simulink model "sm_car_"  (R2026b)
settings: Solver=ode23t  StopTime=100  MaxStep=0.4  AbsTol=1e-3  EnableMultiTasking=on
PreLoadFcn:
  | % Due to usability issue in Repeating Sequence block
  | warning('off','Simulink:Masking:Invalid');
  | 
  | % Eliminate unnecessary warnings in inactive variants
  | % Warnings generated only if you click through inactive variant
  | warning('off','MATLAB:nonExistentField');
  | warning('off','Simulink:Parameters:BlkParamUndefined');
PostLoadFcn:
  | set_param([bdroot '/Vehicle'],'popup_trailer','Off')
  | warning('off','sm:sli:setup:compile:LocalSolverNotSupported')
  | %sm_car_config_maneuver(bdroot,'WOT Braking');
  | sm_car_config_vehicle(bdroot,'false');
  | sm_car_config_logging(bdroot);
InitFcn:
  | sm_car_config_camera;
  | Vehicle = sm_car_vehcfg_checkConfig(Vehicle);
  | sm_car_check_tire_model(bdroot);
StartFcn:
  | tic;
StopFcn:
  | Elapsed_Sim_Time = toc;
  | % disp(['Elapsed Sim Time = ' num2str(Elapsed_Sim_Time)]);
undefined symbols (not defined in the file or in its folder): acc_theta, accel_ramp_rate, Axle1D, AxleIn, Camera, Control, Driver, Init, Maneuver, Pedal, Scene, ShaftL1, ShaftL2, ShaftR1, ShaftR2, Visual, X, xy_data_car_side, Y, Z
libraries: sm_lib x290, fl_lib x171, nesl_utility x144, simulink x60, simulink_extras x14, sdl_lib x14, SimscapeFluids_lib x7, Damper_Element x4, Tire_1x2x x4, ee_lib x3, Scene_Utilities x3, sharedTrackingLibrary x2
(part 7 of 22)

== system sm_car_/Vehicle/Trailer/None ==
  note: Ports deliberately not connected. They are necessary for unit tests, but not necessary here.
  "RdBus " : Inport
  "DrvBus " : Inport  Port=2
  "CtrlBus " : Inport  Port=3
  Ground : Ground
  Reference Frame : sm_lib/Frames and Transforms/Reference Frame
  Terminator : Terminator
  Terminator1 : Terminator
  Terminator2 : Terminator
  " C" : PMIOPort  Side=Left
  " W" : PMIOPort  Port=2  Side=Left
  " Hitch" : PMIOPort  Port=3  Side=Right
  " VehBus" : Outport  VectorParamsAs1DForOutWhenUnconnected=off
  wires:
  "RdBus "/1 -> Terminator/1
  "DrvBus "/1 -> Terminator1/1
  "CtrlBus "/1 -> Terminator2/1
  Ground/1 -> " VehBus"/1
  connections:
  " Hitch"/RConn1 -- Reference Frame/RConn1

== system sm_car_/Vehicle/Vehicle/A1 to World ==
  Body World Joint : sm_lib/Joints/6-DOF Joint  JointMode=Normal  CompositeWrenchDir=FollowerOnBase  CompositeWrenchFrame=BaseFrame  SenseConstraintForce=off  SenseConstraintTorque=off  SenseTotalForce=off  SenseTotalTorque=off  PxPositionTargetSpecify=off  PxPositionTargetPriority=Low  PxPositionTargetValue=Init.sChassis.Value(1)  PxPositionTargetValueUnits=m  PxVelocityTargetSpecify=off  PxVelocityTargetPriority=Low  PxVelocityTargetValue=initial_vveh(1)  PxVelocityTargetValueUnits=m/s  PxEquilibriumPosition=0  PxEquilibriumPositionUnits=m  PxSpringStiffness=0  PxSpringStiffnessUnits=N/m  PxDampingCoefficient=0  PxDampingCoefficientUnits=N/(m/s)  PxLowerLimitSpecify=off  PxLowerLimitBound=-1  PxLowerLimitBoundUnits=m  PxLowerLimitStiffness=1e6  PxLowerLimitStiffnessUnits=N/m  PxLowerLimitDamping=1e3  PxLowerLimitDampingUnits=N/(m/s)  PxLowerLimitTransitionRegionWidth=1e-4  PxLowerLimitTransitionRegionWidthUnits=m  PxUpperLimitSpecify=off  PxUpperLimitBound=1  PxUpperLimitBoundUnits=m  PxUpperLimitStiffness=1e6  PxUpperLimitStiffnessUnits=N/m  PxUpperLimitDamping=1e3  PxUpperLimitDampingUnits=N/(m/s)  PxUpperLimitTransitionRegionWidth=1e-4  PxUpperLimitTransitionRegionWidthUnits=m  PxTorqueActuationMode=NoTorque  PxMotionActuationMode=ComputedMotion  PxSensePosition=off  PxSenseVelocity=off  PxSenseAcceleration=off  PxSenseTorqueForce=off  PxSenseLowerLimitTorqueForce=off  PxSenseUpperLimitTorqueForce=off  PyPositionTargetSpecify=off  PyPositionTargetPriority=Low  PyPositionTargetValue=Init.sChassis.Value(2)  PyPositionTargetValueUnits=m  PyVelocityTargetSpecify=off  PyVelocityTargetPriority=Low  PyVelocityTargetValue=initial_vveh(2)  PyVelocityTargetValueUnits=m/s  PyEquilibriumPosition=0  PyEquilibriumPositionUnits=m  PySpringStiffness=0  PySpringStiffnessUnits=N/m  PyDampingCoefficient=0  PyDampingCoefficientUnits=N/(m/s)  PyLowerLimitSpecify=off  PyLowerLimitBound=-1  PyLowerLimitBoundUnits=m  PyLowerLimitStiffness=1e6  PyLowerLimitStiffnessUnits=N/m  PyLowerLimitDamping=1e3  PyLowerLimitDampingUnits=N/(m/s)  PyLowerLimitTransitionRegionWidth=1e-4  PyLowerLimitTransitionRegionWidthUnits=m  PyUpperLimitSpecify=off  PyUpperLimitBound=1  PyUpperLimitBoundUnits=m  PyUpperLimitStiffness=1e6  PyUpperLimitStiffnessUnits=N/m  PyUpperLimitDamping=1e3  PyUpperLimitDampingUnits=N/(m/s)  PyUpperLimitTransitionRegionWidth=1e-4  PyUpperLimitTransitionRegionWidthUnits=m  PyTorqueActuationMode=NoTorque  PyMotionActuationMode=ComputedMotion  PySensePosition=off  PySenseVelocity=off  PySenseAcceleration=off  PySenseTorqueForce=off  PySenseLowerLimitTorqueForce=off  PySenseUpperLimitTorqueForce=off  PzPositionTargetSpecify=off  PzPositionTargetPriority=Low  PzPositionTargetValue=Init.sChassis.Value(3)  PzPositionTargetValueUnits=m  PzVelocityTargetSpecify=off  PzVelocityTargetPriority=Low  PzVelocityTargetValue=initial_vveh(3)  PzVelocityTargetValueUnits=m/s  PzEquilibriumPosition=0  PzEquilibriumPositionUnits=m  PzSpringStiffness=0  PzSpringStiffnessUnits=N/m  PzDampingCoefficient=0  PzDampingCoefficientUnits=N/(m/s)  PzLowerLimitSpecify=off  PzLowerLimitBound=-1  PzLowerLimitBoundUnits=m  PzLowerLimitStiffness=1e6  PzLowerLimitStiffnessUnits=N/m  PzLowerLimitDamping=1e3  PzLowerLimitDampingUnits=N/(m/s)  PzLowerLimitTransitionRegionWidth=1e-4  PzLowerLimitTransitionRegionWidthUnits=m  PzUpperLimitSpecify=off  PzUpperLimitBound=1  PzUpperLimitBoundUnits=m  PzUpperLimitStiffness=1e6  PzUpperLimitStiffnessUnits=N/m  PzUpperLimitDamping=1e3  PzUpperLimitDampingUnits=N/(m/s)  PzUpperLimitTransitionRegionWidth=1e-4  PzUpperLimitTransitionRegionWidthUnits=m  PzTorqueActuationMode=NoTorque  PzMotionActuationMode=ComputedMotion  PzSensePosition=on  PzSenseVelocity=off  PzSenseAcceleration=off  PzSenseTorqueForce=off  PzSenseLowerLimitTorqueForce=off  PzSenseUpperLimitTorqueForce=off  SphPositionTargetSpecify=off  SphPositionTargetPriority=Low  SphPositionTargetRotationMethod=RotationSequence  SphPositionTargetFollAlignAxisA=+X  SphPositionTargetBaseAlignAxisA=+Y  SphPositionTargetFollAlignAxisB=+Y  SphPositionTargetBaseAlignAxisB=+Z  SphPositionTargetRotationStandardAxis=+Z  SphPositionTargetRotationAngle=0.0  SphPositionTargetRotationAngleUnits=deg  SphPositionTargetRotationArbitraryAxis=[0 0 1]  SphPositionTargetRotationSequenceAxes=FollowerAxes  SphPositionTargetRotationSequence=ZYX  SphPositionTargetRotationSequenceAngles=initial_aveh  SphPositionTargetRotationSequenceAnglesUnits=rad  SphPositionTargetRotationMatrix=[1 0 0; 0 1 0; 0 0 1]  SphPositionTargetQuaternion=[1 0 0 0]  SphVelocityTargetSpecify=off  SphVelocityTargetPriority=High  SphVelocityTargetValue=[0 0 0]  SphVelocityTargetValueUnits=deg/s  SphVelocityTargetInFollowerFrame=on  SphEqPosRotationMethod=None  SphEqPosFollAlignAxisA=+X  SphEqPosBaseAlignAxisA=+Y  SphEqPosFollAlignAxisB=+Y  SphEqPosBaseAlignAxisB=+Z  SphEqPosRotationStandardAxis=+Z  SphEqPosRotationAngle=0.0  SphEqPosRotationAngleUnits=deg  SphEqPosRotationArbitraryAxis=[0 0 1]  SphEqPosRotationSequenceAxes=FollowerAxes  SphEqPosRotationSequence=XYX  SphEqPosRotationSequenceAngles=[0 0 0]  SphEqPosRotationSequenceAnglesUnits=deg  SphEqPosRotationMatrix=[1 0 0; 0 1 0; 0 0 1]  SphEqPosQuaternion=[1 0 0 0]  SphSpringStiffness=0  SphSpringStiffnessUnits=N*m/deg  SphDampingCoefficient=0  SphDampingCoefficientUnits=N*m/(deg/s)  SphLowerLimitSpecify=off  SphLowerLimitBound=15  SphLowerLimitBoundUnits=deg  SphLowerLimitStiffness=1e4  SphLowerLimitStiffnessUnits=N*m/deg  SphLowerLimitDamping=10  SphLowerLimitDampingUnits=N*m/(deg/s)  SphLowerLimitTransitionRegionWidth=0.1  SphLowerLimitTransitionRegionWidthUnits=deg  SphUpperLimitSpecify=off  SphUpperLimitBound=45  SphUpperLimitBoundUnits=deg  SphUpperLimitStiffness=1e4  SphUpperLimitStiffnessUnits=N*m/deg  SphUpperLimitDamping=10  SphUpperLimitDampingUnits=N*m/(deg/s)  SphUpperLimitTransitionRegionWidth=0.1  SphUpperLimitTransitionRegionWidthUnits=deg  SphTorqueActuationMode=NoTorque  SphActuateTorqueX=off  SphActuateTorqueY=off  SphActuateTorqueZ=off  SphActuateTorque=off  SphActuationFrame=BaseFrame  SphSensePosition=off  SphSenseVelocityX=off  SphSenseVelocityY=off  SphSenseVelocityZ=off  SphSenseVelocity=off  SphSenseAccelerationX=off  SphSenseAccelerationY=off  SphSenseAccelerationZ=off  SphSenseAcceleration=off  SphSenseLowerLimitTorqueMag=off  SphSenseUpperLimitTorqueMag=off  SphSensingFrame=BaseFrame
  PS-Simulink Converter2 : nesl_utility/PS-Simulink Converter  PhysicalDomain=network_engine_domain  SubClassName=ps_output  LeftPortType=input  RightPortType=output  PseudoPeriodic=off  Frequencies=[]  VectorFormat=1-D array  Unit=m  AffineConversion=off
  Transform Sensor : sm_lib/Frames and Transforms/Transform Sensor  ObservationFrame=World  ExpressedInFrame=World  RotationSequence=XYX  SenseAngle=off  SenseAxis=off  SenseQ=off  SenseR=off  SenseRotationSequence=off  SenseOmegaX=off  SenseOmegaY=off  SenseOmegaZ=off  SenseOmega=off  SenseQDot=off  SenseRDot=off  SenseRotationSequenceDot=off  SenseAlphaX=off  SenseAlphaY=off  SenseAlphaZ=off  SenseAlpha=off  SenseQDDot=off  SenseRDDot=off  SenseX=off  SenseY=off  SenseZ=off  SenseXYZ=off  SenseRad=off  SenseAzim=off  SenseDist=off  SenseInc=off  SenseXDot=off  SenseYDot=off  SenseZDot=off  SenseXYZDot=off  SenseRadDot=off  SenseAzimDot=off  SenseDistDot=off  SenseIncDot=off  SenseXDDot=off  SenseYDDot=off  SenseZDDot=off  SenseXYZDDot=off  SenseRadDDot=off  SenseAzimDDot=off  SenseDistDDot=off  SenseIncDDot=off
  F : PMIOPort  Side=Left
  B : PMIOPort  Port=2  Side=Right
  Bus Element Out6 : Outport  VectorParamsAs1DForOutWhenUnconnected=off  PortName=World  Element=z
  wires:
  PS-Simulink Converter2/1 -> Bus Element Out6/1
  connections:
  Body World Joint/RConn2 -- PS-Simulink Converter2/LConn1
  Body World Joint/RConn1 -- F/RConn1 -- Transform Sensor/RConn1
  Body World Joint/LConn1 -- B/RConn1 -- Transform Sensor/LConn1

== system sm_car_/Vehicle/Vehicle/A2 to World ==
  Body World Joint : sm_lib/Joints/6-DOF Joint  JointMode=Normal  CompositeWrenchDir=FollowerOnBase  CompositeWrenchFrame=BaseFrame  SenseConstraintForce=off  SenseConstraintTorque=off  SenseTotalForce=off  SenseTotalTorque=off  PxPositionTargetSpecify=off  PxPositionTargetPriority=Low  PxPositionTargetValue=Init.sChassis.Value(1)  PxPositionTargetValueUnits=m  PxVelocityTargetSpecify=off  PxVelocityTargetPriority=Low  PxVelocityTargetValue=initial_vveh(1)  PxVelocityTargetValueUnits=m/s  PxEquilibriumPosition=0  PxEquilibriumPositionUnits=m  PxSpringStiffness=0  PxSpringStiffnessUnits=N/m  PxDampingCoefficient=0  PxDampingCoefficientUnits=N/(m/s)  PxLowerLimitSpecify=off  PxLowerLimitBound=-1  PxLowerLimitBoundUnits=m  PxLowerLimitStiffness=1e6  PxLowerLimitStiffnessUnits=N/m  PxLowerLimitDamping=1e3  PxLowerLimitDampingUnits=N/(m/s)  PxLowerLimitTransitionRegionWidth=1e-4  PxLowerLimitTransitionRegionWidthUnits=m  PxUpperLimitSpecify=off  PxUpperLimitBound=1  PxUpperLimitBoundUnits=m  PxUpperLimitStiffness=1e6  PxUpperLimitStiffnessUnits=N/m  PxUpperLimitDamping=1e3  PxUpperLimitDampingUnits=N/(m/s)  PxUpperLimitTransitionRegionWidth=1e-4  PxUpperLimitTransitionRegionWidthUnits=m  PxTorqueActuationMode=NoTorque  PxMotionActuationMode=ComputedMotion  PxSensePosition=off  PxSenseVelocity=off  PxSenseAcceleration=off  PxSenseTorqueForce=off  PxSenseLowerLimitTorqueForce=off  PxSenseUpperLimitTorqueForce=off  PyPositionTargetSpecify=off  PyPositionTargetPriority=Low  PyPositionTargetValue=Init.sChassis.Value(2)  PyPositionTargetValueUnits=m  PyVelocityTargetSpecify=off  PyVelocityTargetPriority=Low  PyVelocityTargetValue=initial_vveh(2)  PyVelocityTargetValueUnits=m/s  PyEquilibriumPosition=0  PyEquilibriumPositionUnits=m  PySpringStiffness=0  PySpringStiffnessUnits=N/m  PyDampingCoefficient=0  PyDampingCoefficientUnits=N/(m/s)  PyLowerLimitSpecify=off  PyLowerLimitBound=-1  PyLowerLimitBoundUnits=m  PyLowerLimitStiffness=1e6  PyLowerLimitStiffnessUnits=N/m  PyLowerLimitDamping=1e3  PyLowerLimitDampingUnits=N/(m/s)  PyLowerLimitTransitionRegionWidth=1e-4  PyLowerLimitTransitionRegionWidthUnits=m  PyUpperLimitSpecify=off  PyUpperLimitBound=1  PyUpperLimitBoundUnits=m  PyUpperLimitStiffness=1e6  PyUpperLimitStiffnessUnits=N/m  PyUpperLimitDamping=1e3  PyUpperLimitDampingUnits=N/(m/s)  PyUpperLimitTransitionRegionWidth=1e-4  PyUpperLimitTransitionRegionWidthUnits=m  PyTorqueActuationMode=NoTorque  PyMotionActuationMode=ComputedMotion  PySensePosition=off  PySenseVelocity=off  PySenseAcceleration=off  PySenseTorqueForce=off  PySenseLowerLimitTorqueForce=off  PySenseUpperLimitTorqueForce=off  PzPositionTargetSpecify=off  PzPositionTargetPriority=Low  PzPositionTargetValue=Init.sChassis.Value(3)  PzPositionTargetValueUnits=m  PzVelocityTargetSpecify=off  PzVelocityTargetPriority=Low  PzVelocityTargetValue=initial_vveh(3)  PzVelocityTargetValueUnits=m/s  PzEquilibriumPosition=0  PzEquilibriumPositionUnits=m  PzSpringStiffness=0  PzSpringStiffnessUnits=N/m  PzDampingCoefficient=0  PzDampingCoefficientUnits=N/(m/s)  PzLowerLimitSpecify=off  PzLowerLimitBound=-1  PzLowerLimitBoundUnits=m  PzLowerLimitStiffness=1e6  PzLowerLimitStiffnessUnits=N/m  PzLowerLimitDamping=1e3  PzLowerLimitDampingUnits=N/(m/s)  PzLowerLimitTransitionRegionWidth=1e-4  PzLowerLimitTransitionRegionWidthUnits=m  PzUpperLimitSpecify=off  PzUpperLimitBound=1  PzUpperLimitBoundUnits=m  PzUpperLimitStiffness=1e6  PzUpperLimitStiffnessUnits=N/m  PzUpperLimitDamping=1e3  PzUpperLimitDampingUnits=N/(m/s)  PzUpperLimitTransitionRegionWidth=1e-4  PzUpperLimitTransitionRegionWidthUnits=m  PzTorqueActuationMode=NoTorque  PzMotionActuationMode=ComputedMotion  PzSensePosition=on  PzSenseVelocity=off  PzSenseAcceleration=off  PzSenseTorqueForce=off  PzSenseLowerLimitTorqueForce=off  PzSenseUpperLimitTorqueForce=off  SphPositionTargetSpecify=off  SphPositionTargetPriority=Low  SphPositionTargetRotationMethod=RotationSequence  SphPositionTargetFollAlignAxisA=+X  SphPositionTargetBaseAlignAxisA=+Y  SphPositionTargetFollAlignAxisB=+Y  SphPositionTargetBaseAlignAxisB=+Z  SphPositionTargetRotationStandardAxis=+Z  SphPositionTargetRotationAngle=0.0  SphPositionTargetRotationAngleUnits=deg  SphPositionTargetRotationArbitraryAxis=[0 0 1]  SphPositionTargetRotationSequenceAxes=FollowerAxes  SphPositionTargetRotationSequence=ZYX  SphPositionTargetRotationSequenceAngles=initial_aveh  SphPositionTargetRotationSequenceAnglesUnits=rad  SphPositionTargetRotationMatrix=[1 0 0; 0 1 0; 0 0 1]  SphPositionTargetQuaternion=[1 0 0 0]  SphVelocityTargetSpecify=off  SphVelocityTargetPriority=High  SphVelocityTargetValue=[0 0 0]  SphVelocityTargetValueUnits=deg/s  SphVelocityTargetInFollowerFrame=on  SphEqPosRotationMethod=None  SphEqPosFollAlignAxisA=+X  SphEqPosBaseAlignAxisA=+Y  SphEqPosFollAlignAxisB=+Y  SphEqPosBaseAlignAxisB=+Z  SphEqPosRotationStandardAxis=+Z  SphEqPosRotationAngle=0.0  SphEqPosRotationAngleUnits=deg  SphEqPosRotationArbitraryAxis=[0 0 1]  SphEqPosRotationSequenceAxes=FollowerAxes  SphEqPosRotationSequence=XYX  SphEqPosRotationSequenceAngles=[0 0 0]  SphEqPosRotationSequenceAnglesUnits=deg  SphEqPosRotationMatrix=[1 0 0; 0 1 0; 0 0 1]  SphEqPosQuaternion=[1 0 0 0]  SphSpringStiffness=0  SphSpringStiffnessUnits=N*m/deg  SphDampingCoefficient=0  SphDampingCoefficientUnits=N*m/(deg/s)  SphLowerLimitSpecify=off  SphLowerLimitBound=15  SphLowerLimitBoundUnits=deg  SphLowerLimitStiffness=1e4  SphLowerLimitStiffnessUnits=N*m/deg  SphLowerLimitDamping=10  SphLowerLimitDampingUnits=N*m/(deg/s)  SphLowerLimitTransitionRegionWidth=0.1  SphLowerLimitTransitionRegionWidthUnits=deg  SphUpperLimitSpecify=off  SphUpperLimitBound=45  SphUpperLimitBoundUnits=deg  SphUpperLimitStiffness=1e4  SphUpperLimitStiffnessUnits=N*m/deg  SphUpperLimitDamping=10  SphUpperLimitDampingUnits=N*m/(deg/s)  SphUpperLimitTransitionRegionWidth=0.1  SphUpperLimitTransitionRegionWidthUnits=deg  SphTorqueActuationMode=NoTorque  SphActuateTorqueX=off  SphActuateTorqueY=off  SphActuateTorqueZ=off  SphActuateTorque=off  SphActuationFrame=BaseFrame  SphSensePosition=off  SphSenseVelocityX=off  SphSenseVelocityY=off  SphSenseVelocityZ=off  SphSenseVelocity=off  SphSenseAccelerationX=off  SphSenseAccelerationY=off  SphSenseAccelerationZ=off  SphSenseAcceleration=off  SphSenseLowerLimitTorqueMag=off  SphSenseUpperLimitTorqueMag=off  SphSensingFrame=BaseFrame
  PS-Simulink Converter2 : nesl_utility/PS-Simulink Converter  PhysicalDomain=network_engine_domain  SubClassName=ps_output  LeftPortType=input  RightPortType=output  PseudoPeriodic=off  Frequencies=[]  VectorFormat=1-D array  Unit=m  AffineConversion=off
  Transform Sensor : sm_lib/Frames and Transforms/Transform Sensor  ObservationFrame=World  ExpressedInFrame=World  RotationSequence=XYX  SenseAngle=off  SenseAxis=off  SenseQ=off  SenseR=off  SenseRotationSequence=off  SenseOmegaX=off  SenseOmegaY=off  SenseOmegaZ=off  SenseOmega=off  SenseQDot=off  SenseRDot=off  SenseRotationSequenceDot=off  SenseAlphaX=off  SenseAlphaY=off  SenseAlphaZ=off  SenseAlpha=off  SenseQDDot=off  SenseRDDot=off  SenseX=off  SenseY=off  SenseZ=off  SenseXYZ=off  SenseRad=off  SenseAzim=off  SenseDist=off  SenseInc=off  SenseXDot=off  SenseYDot=off  SenseZDot=off  SenseXYZDot=off  SenseRadDot=off  SenseAzimDot=off  SenseDistDot=off  SenseIncDot=off  SenseXDDot=off  SenseYDDot=off  SenseZDDot=off  SenseXYZDDot=off  SenseRadDDot=off  SenseAzimDDot=off  SenseDistDDot=off  SenseIncDDot=off
  F : PMIOPort  Side=Left
  B : PMIOPort  Port=2  Side=Right
  Bus Element Out6 : Outport  VectorParamsAs1DForOutWhenUnconnected=off  PortName=World  Element=z
  wires:
  PS-Simulink Converter2/1 -> Bus Element Out6/1
  connections:
  B/RConn1 -- Transform Sensor/LConn1 -- Body World Joint/LConn1
  Body World Joint/RConn1 -- Transform Sensor/RConn1 -- F/RConn1
  Body World Joint/RConn2 -- PS-Simulink Converter2/LConn1

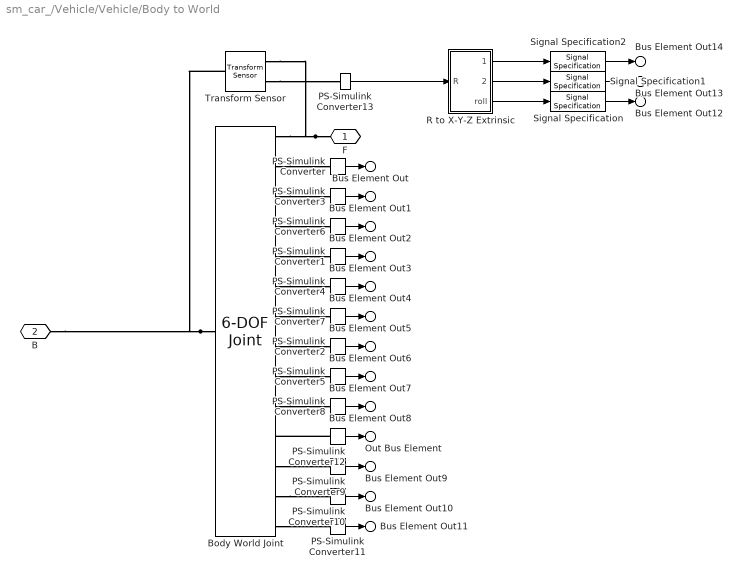
== system sm_car_/Vehicle/Vehicle/Body to World ==
  Body World Joint : sm_lib/Joints/6-DOF Joint  JointMode=Normal  CompositeWrenchDir=FollowerOnBase  CompositeWrenchFrame=BaseFrame  SenseConstraintForce=off  SenseConstraintTorque=off  SenseTotalForce=off  SenseTotalTorque=off  PxPositionTargetSpecify=on  PxPositionTargetPriority=Low  PxPositionTargetValue=Init.sChassis.Value(1)  PxPositionTargetValueUnits=m  PxVelocityTargetSpecify=on  PxVelocityTargetPriority=Low  PxVelocityTargetValue=initial_vveh(1)  PxVelocityTargetValueUnits=m/s  PxEquilibriumPosition=0  PxEquilibriumPositionUnits=m  PxSpringStiffness=0  PxSpringStiffnessUnits=N/m  PxDampingCoefficient=0  PxDampingCoefficientUnits=N/(m/s)  PxLowerLimitSpecify=off  PxLowerLimitBound=-1  PxLowerLimitBoundUnits=m  PxLowerLimitStiffness=1e6  PxLowerLimitStiffnessUnits=N/m  PxLowerLimitDamping=1e3  PxLowerLimitDampingUnits=N/(m/s)  PxLowerLimitTransitionRegionWidth=1e-4  PxLowerLimitTransitionRegionWidthUnits=m  PxUpperLimitSpecify=off  PxUpperLimitBound=1  PxUpperLimitBoundUnits=m  PxUpperLimitStiffness=1e6  PxUpperLimitStiffnessUnits=N/m  PxUpperLimitDamping=1e3  PxUpperLimitDampingUnits=N/(m/s)  PxUpperLimitTransitionRegionWidth=1e-4  PxUpperLimitTransitionRegionWidthUnits=m  PxTorqueActuationMode=NoTorque  PxMotionActuationMode=ComputedMotion  PxSensePosition=on  PxSenseVelocity=on  PxSenseAcceleration=on  PxSenseTorqueForce=off  PxSenseLowerLimitTorqueForce=off  PxSenseUpperLimitTorqueForce=off  PyPositionTargetSpecify=on  PyPositionTargetPriority=Low  PyPositionTargetValue=Init.sChassis.Value(2)  PyPositionTargetValueUnits=m  PyVelocityTargetSpecify=on  PyVelocityTargetPriority=Low  PyVelocityTargetValue=initial_vveh(2)  PyVelocityTargetValueUnits=m/s  PyEquilibriumPosition=0  PyEquilibriumPositionUnits=m  PySpringStiffness=0  PySpringStiffnessUnits=N/m  PyDampingCoefficient=0  PyDampingCoefficientUnits=N/(m/s)  PyLowerLimitSpecify=off  PyLowerLimitBound=-1  PyLowerLimitBoundUnits=m  PyLowerLimitStiffness=1e6  PyLowerLimitStiffnessUnits=N/m  PyLowerLimitDamping=1e3  PyLowerLimitDampingUnits=N/(m/s)  PyLowerLimitTransitionRegionWidth=1e-4  PyLowerLimitTransitionRegionWidthUnits=m  PyUpperLimitSpecify=off  PyUpperLimitBound=1  PyUpperLimitBoundUnits=m  PyUpperLimitStiffness=1e6  PyUpperLimitStiffnessUnits=N/m  PyUpperLimitDamping=1e3  PyUpperLimitDampingUnits=N/(m/s)  PyUpperLimitTransitionRegionWidth=1e-4  PyUpperLimitTransitionRegionWidthUnits=m  PyTorqueActuationMode=NoTorque  PyMotionActuationMode=ComputedMotion  PySensePosition=on  PySenseVelocity=on  PySenseAcceleration=on  PySenseTorqueForce=off  PySenseLowerLimitTorqueForce=off  PySenseUpperLimitTorqueForce=off  PzPositionTargetSpecify=on  PzPositionTargetPriority=Low  PzPositionTargetValue=Init.sChassis.Value(3)  PzPositionTargetValueUnits=m  PzVelocityTargetSpecify=on  PzVelocityTargetPriority=Low  PzVelocityTargetValue=initial_vveh(3)  PzVelocityTargetValueUnits=m/s  PzEquilibriumPosition=0  PzEquilibriumPositionUnits=m  PzSpringStiffness=0  PzSpringStiffnessUnits=N/m  PzDampingCoefficient=0  PzDampingCoefficientUnits=N/(m/s)  PzLowerLimitSpecify=off  PzLowerLimitBound=-1  PzLowerLimitBoundUnits=m  PzLowerLimitStiffness=1e6  PzLowerLimitStiffnessUnits=N/m  PzLowerLimitDamping=1e3  PzLowerLimitDampingUnits=N/(m/s)  PzLowerLimitTransitionRegionWidth=1e-4  PzLowerLimitTransitionRegionWidthUnits=m  PzUpperLimitSpecify=off  PzUpperLimitBound=1  PzUpperLimitBoundUnits=m  PzUpperLimitStiffness=1e6  PzUpperLimitStiffnessUnits=N/m  PzUpperLimitDamping=1e3  PzUpperLimitDampingUnits=N/(m/s)  PzUpperLimitTransitionRegionWidth=1e-4  PzUpperLimitTransitionRegionWidthUnits=m  PzTorqueActuationMode=NoTorque  PzMotionActuationMode=ComputedMotion  PzSensePosition=on  PzSenseVelocity=on  PzSenseAcceleration=on  PzSenseTorqueForce=off  PzSenseLowerLimitTorqueForce=off  PzSenseUpperLimitTorqueForce=off  SphPositionTargetSpecify=on  SphPositionTargetPriority=Low  SphPositionTargetRotationMethod=RotationSequence  SphPositionTargetFollAlignAxisA=+X  SphPositionTargetBaseAlignAxisA=+Y  SphPositionTargetFollAlignAxisB=+Y  SphPositionTargetBaseAlignAxisB=+Z  SphPositionTargetRotationStandardAxis=+Z  SphPositionTargetRotationAngle=0.0  SphPositionTargetRotationAngleUnits=deg  SphPositionTargetRotationArbitraryAxis=[0 0 1]  SphPositionTargetRotationSequenceAxes=FollowerAxes  SphPositionTargetRotationSequence=ZYX  SphPositionTargetRotationSequenceAngles=initial_aveh  SphPositionTargetRotationSequenceAnglesUnits=rad  SphPositionTargetRotationMatrix=[1 0 0; 0 1 0; 0 0 1]  SphPositionTargetQuaternion=[1 0 0 0]  SphVelocityTargetSpecify=off  SphVelocityTargetPriority=High  SphVelocityTargetValue=[0 0 0]  SphVelocityTargetValueUnits=deg/s  SphVelocityTargetInFollowerFrame=on  SphEqPosRotationMethod=None  SphEqPosFollAlignAxisA=+X  SphEqPosBaseAlignAxisA=+Y  SphEqPosFollAlignAxisB=+Y  SphEqPosBaseAlignAxisB=+Z  SphEqPosRotationStandardAxis=+Z  SphEqPosRotationAngle=0.0  SphEqPosRotationAngleUnits=deg  SphEqPosRotationArbitraryAxis=[0 0 1]  SphEqPosRotationSequenceAxes=FollowerAxes  SphEqPosRotationSequence=XYX  SphEqPosRotationSequenceAngles=[0 0 0]  SphEqPosRotationSequenceAnglesUnits=deg  SphEqPosRotationMatrix=[1 0 0; 0 1 0; 0 0 1]  SphEqPosQuaternion=[1 0 0 0]  SphSpringStiffness=0  SphSpringStiffnessUnits=N*m/deg  SphDampingCoefficient=0  SphDampingCoefficientUnits=N*m/(deg/s)  SphLowerLimitSpecify=off  SphLowerLimitBound=15  SphLowerLimitBoundUnits=deg  SphLowerLimitStiffness=1e4  SphLowerLimitStiffnessUnits=N*m/deg  SphLowerLimitDamping=10  SphLowerLimitDampingUnits=N*m/(deg/s)  SphLowerLimitTransitionRegionWidth=0.1  SphLowerLimitTransitionRegionWidthUnits=deg  SphUpperLimitSpecify=off  SphUpperLimitBound=45  SphUpperLimitBoundUnits=deg  SphUpperLimitStiffness=1e4  SphUpperLimitStiffnessUnits=N*m/deg  SphUpperLimitDamping=10  SphUpperLimitDampingUnits=N*m/(deg/s)  SphUpperLimitTransitionRegionWidth=0.1  SphUpperLimitTransitionRegionWidthUnits=deg  SphTorqueActuationMode=NoTorque  SphActuateTorqueX=off  SphActuateTorqueY=off  SphActuateTorqueZ=off  SphActuateTorque=off  SphActuationFrame=BaseFrame  SphSensePosition=on  SphSenseVelocityX=on  SphSenseVelocityY=on  SphSenseVelocityZ=on  SphSenseVelocity=off  SphSenseAccelerationX=off  SphSenseAccelerationY=off  SphSenseAccelerationZ=off  SphSenseAcceleration=off  SphSenseLowerLimitTorqueMag=off  SphSenseUpperLimitTorqueMag=off  SphSensingFrame=BaseFrame
  PS-Simulink Converter : nesl_utility/PS-Simulink Converter  PhysicalDomain=network_engine_domain  SubClassName=ps_output  LeftPortType=input  RightPortType=output  PseudoPeriodic=off  Frequencies=[]  VectorFormat=1-D array  Unit=m  AffineConversion=off
  PS-Simulink Converter1 : nesl_utility/PS-Simulink Converter  PhysicalDomain=network_engine_domain  SubClassName=ps_output  LeftPortType=input  RightPortType=output  PseudoPeriodic=off  Frequencies=[]  VectorFormat=1-D array  Unit=m  AffineConversion=off
  PS-Simulink Converter10 : nesl_utility/PS-Simulink Converter  PhysicalDomain=network_engine_domain  SubClassName=ps_output  LeftPortType=input  RightPortType=output  PseudoPeriodic=off  Frequencies=[]  VectorFormat=1-D array  Unit=rad/s  AffineConversion=off
  PS-Simulink Converter11 : nesl_utility/PS-Simulink Converter  PhysicalDomain=network_engine_domain  SubClassName=ps_output  LeftPortType=input  RightPortType=output  PseudoPeriodic=off  Frequencies=[]  VectorFormat=1-D array  Unit=rad/s  AffineConversion=off
  PS-Simulink Converter12 : nesl_utility/PS-Simulink Converter  PhysicalDomain=network_engine_domain  SubClassName=ps_output  LeftPortType=input  RightPortType=output  PseudoPeriodic=off  Frequencies=[]  VectorFormat=1-D array  Unit=1  AffineConversion=off
  PS-Simulink Converter13 : nesl_utility/PS-Simulink Converter  PhysicalDomain=network_engine_domain  SubClassName=ps_output  LeftPortType=input  RightPortType=output  PseudoPeriodic=off  Frequencies=[]  VectorFormat=1-D array  Unit=1  AffineConversion=off
  PS-Simulink Converter2 : nesl_utility/PS-Simulink Converter  PhysicalDomain=network_engine_domain  SubClassName=ps_output  LeftPortType=input  RightPortType=output  PseudoPeriodic=off  Frequencies=[]  VectorFormat=1-D array  Unit=m  AffineConversion=off
  PS-Simulink Converter3 : nesl_utility/PS-Simulink Converter  PhysicalDomain=network_engine_domain  SubClassName=ps_output  LeftPortType=input  RightPortType=output  PseudoPeriodic=off  Frequencies=[]  VectorFormat=1-D array  Unit=m/s  AffineConversion=off
  PS-Simulink Converter4 : nesl_utility/PS-Simulink Converter  PhysicalDomain=network_engine_domain  SubClassName=ps_output  LeftPortType=input  RightPortType=output  PseudoPeriodic=off  Frequencies=[]  VectorFormat=1-D array  Unit=m/s  AffineConversion=off
  PS-Simulink Converter5 : nesl_utility/PS-Simulink Converter  PhysicalDomain=network_engine_domain  SubClassName=ps_output  LeftPortType=input  RightPortType=output  PseudoPeriodic=off  Frequencies=[]  VectorFormat=1-D array  Unit=m/s  AffineConversion=off
  PS-Simulink Converter6 : nesl_utility/PS-Simulink Converter  PhysicalDomain=network_engine_domain  SubClassName=ps_output  LeftPortType=input  RightPortType=output  PseudoPeriodic=off  Frequencies=[]  VectorFormat=1-D array  Unit=m/s^2  AffineConversion=off
  PS-Simulink Converter7 : nesl_utility/PS-Simulink Converter  PhysicalDomain=network_engine_domain  SubClassName=ps_output  LeftPortType=input  RightPortType=output  PseudoPeriodic=off  Frequencies=[]  VectorFormat=1-D array  Unit=m/s^2  AffineConversion=off
  PS-Simulink Converter8 : nesl_utility/PS-Simulink Converter  PhysicalDomain=network_engine_domain  SubClassName=ps_output  LeftPortType=input  RightPortType=output  PseudoPeriodic=off  Frequencies=[]  VectorFormat=1-D array  Unit=m/s^2  AffineConversion=off
  PS-Simulink Converter9 : nesl_utility/PS-Simulink Converter  PhysicalDomain=network_engine_domain  SubClassName=ps_output  LeftPortType=input  RightPortType=output  PseudoPeriodic=off  Frequencies=[]  VectorFormat=1-D array  Unit=rad/s  AffineConversion=off
  R to X-Y-Z Extrinsic : Subsystem  mask(Rotation Matrix to X-Y-Z Extrinsic){}
      mask help: Computes roll / pitch / yaw values assuming they correspond to X, Y, and Z rotations, applied in that order and using extrinsic rotations (rotations applied about the fixed axes of the base frame). Does not handle case where Y (pitch) rotation is +/-90 degrees.
  Signal Specification : SignalSpecification  Unit=rad
  Signal Specification1 : SignalSpecification  Unit=rad
  Signal Specification2 : SignalSpecification  Unit=rad
  Transform Sensor : sm_lib/Frames and Transforms/Transform Sensor  ObservationFrame=World  ExpressedInFrame=World  RotationSequence=XYX  SenseAngle=off  SenseAxis=off  SenseQ=off  SenseR=on  SenseRotationSequence=off  SenseOmegaX=off  SenseOmegaY=off  SenseOmegaZ=off  SenseOmega=off  SenseQDot=off  SenseRDot=off  SenseRotationSequenceDot=off  SenseAlphaX=off  SenseAlphaY=off  SenseAlphaZ=off  SenseAlpha=off  SenseQDDot=off  SenseRDDot=off  SenseX=off  SenseY=off  SenseZ=off  SenseXYZ=off  SenseRad=off  SenseAzim=off  SenseDist=off  SenseInc=off  SenseXDot=off  SenseYDot=off  SenseZDot=off  SenseXYZDot=off  SenseRadDot=off  SenseAzimDot=off  SenseDistDot=off  SenseIncDot=off  SenseXDDot=off  SenseYDDot=off  SenseZDDot=off  SenseXYZDDot=off  SenseRadDDot=off  SenseAzimDDot=off  SenseDistDDot=off  SenseIncDDot=off
  F : PMIOPort  Side=Left
  B : PMIOPort  Port=2  Side=Right
  Bus Element Out : Outport  VectorParamsAs1DForOutWhenUnconnected=off  PortName=World  Element=x
  Bus Element Out3 : Outport  VectorParamsAs1DForOutWhenUnconnected=off  PortName=World  Element=y
  Bus Element Out6 : Outport  VectorParamsAs1DForOutWhenUnconnected=off  PortName=World  Element=z
  Bus Element Out1 : Outport  VectorParamsAs1DForOutWhenUnconnected=off  PortName=World  Element=vx
  Bus Element Out4 : Outport  VectorParamsAs1DForOutWhenUnconnected=off  PortName=World  Element=vy
  Bus Element Out7 : Outport  VectorParamsAs1DForOutWhenUnconnected=off  PortName=World  Element=vz
  Bus Element Out2 : Outport  VectorParamsAs1DForOutWhenUnconnected=off  PortName=World  Element=gx
  Bus Element Out5 : Outport  VectorParamsAs1DForOutWhenUnconnected=off  PortName=World  Element=gy
  Bus Element Out8 : Outport  VectorParamsAs1DForOutWhenUnconnected=off  PortName=World  Element=gz
  Bus Element Out9 : Outport  VectorParamsAs1DForOutWhenUnconnected=off  PortName=World  Element=nRoll
  Bus Element Out10 : Outport  VectorParamsAs1DForOutWhenUnconnected=off  PortName=World  Element=nPitch
  Bus Element Out11 : Outport  VectorParamsAs1DForOutWhenUnconnected=off  PortName=World  Element=nYaw
  Bus Element Out12 : Outport  VectorParamsAs1DForOutWhenUnconnected=off  PortName=World  Element=aRoll
  Bus Element Out13 : Outport  VectorParamsAs1DForOutWhenUnconnected=off  PortName=World  Element=aPitch
  Bus Element Out14 : Outport  VectorParamsAs1DForOutWhenUnconnected=off  PortName=World  Element=aYaw
  Out Bus Element : Outport  VectorParamsAs1DForOutWhenUnconnected=off  PortName=World  Element=Q
  wires:
  R to X-Y-Z Extrinsic/1(yaw) -> Signal Specification2/1
  R to X-Y-Z Extrinsic/3(roll) -> Signal Specification/1
  R to X-Y-Z Extrinsic/2(pitch) -> Signal Specification1/1
  PS-Simulink Converter13/1 -> R to X-Y-Z Extrinsic/1(R)
  PS-Simulink Converter12/1 -> Out Bus Element/1
  PS-Simulink Converter11/1 -> Bus Element Out11/1
  PS-Simulink Converter10/1 -> Bus Element Out10/1
  Signal Specification/1 -> Bus Element Out12/1
  Signal Specification1/1 -> Bus Element Out13/1
  Signal Specification2/1 -> Bus Element Out14/1
  PS-Simulink Converter3/1 -> Bus Element Out1/1
  PS-Simulink Converter2/1 -> Bus Element Out6/1
  PS-Simulink Converter6/1 -> Bus Element Out2/1
  PS-Simulink Converter4/1 -> Bus Element Out4/1
  PS-Simulink Converter/1 -> Bus Element Out/1
  PS-Simulink Converter5/1 -> Bus Element Out7/1
  PS-Simulink Converter9/1 -> Bus Element Out9/1
  PS-Simulink Converter8/1 -> Bus Element Out8/1
  PS-Simulink Converter7/1 -> Bus Element Out5/1
  PS-Simulink Converter1/1 -> Bus Element Out3/1
  connections:
  Transform Sensor/RConn2 -- PS-Simulink Converter13/LConn1
  PS-Simulink Converter12/LConn1 -- Body World Joint/RConn11
  Body World Joint/RConn8 -- PS-Simulink Converter2/LConn1
  Body World Joint/RConn9 -- PS-Simulink Converter5/LConn1
  F/RConn1 -- Transform Sensor/RConn1 -- Body World Joint/RConn1
  Body World Joint/RConn3 -- PS-Simulink Converter3/LConn1
  Body World Joint/RConn10 -- PS-Simulink Converter8/LConn1
  Body World Joint/RConn4 -- PS-Simulink Converter6/LConn1
  Body World Joint/RConn2 -- PS-Simulink Converter/LConn1
  Body World Joint/RConn7 -- PS-Simulink Converter7/LConn1
  Body World Joint/RConn13 -- PS-Simulink Converter10/LConn1
  Body World Joint/RConn14 -- PS-Simulink Converter11/LConn1
  Body World Joint/RConn5 -- PS-Simulink Converter1/LConn1
  Body World Joint/LConn1 -- B/RConn1 -- Transform Sensor/LConn1
  Body World Joint/RConn12 -- PS-Simulink Converter9/LConn1
  Body World Joint/RConn6 -- PS-Simulink Converter4/LConn1

== system sm_car_/Vehicle/Vehicle/Brakes ==
  "DrvBus " : Inport
  "CtrlBus " : Inport  Port=2
  PedalAbstract DiscDisc : Subsystem  Tag=PublishSubsystem  VariantControl=PedalAbstract_DiscDisc  mask(Disc Brakes, Pedal Input){brk_pad_rad_a1=Brakes.Axle1.DiscAndPad.lMeanRadius.Value, brk_pad_rad_a2=Brakes.Axle2.DiscAndPad.lMeanRadius.Value, brk_cyl_bore_a1=Brakes.Axle1.Caliper.lCylinderDiameter.Value, brk_cyl_bore_a2=Brakes.Axle2.Caliper.lCylinderDiameter.Value, brk_n_pads_a1=Brakes.Axle1.DiscAndPad.NPads.Value, brk_n_pads_a2=Brakes.Axle2.DiscAndPad.NPads.Value, brk_mu_static_a1=Brakes.Axle1.DiscAndPad.rMuStatic.Value, brk_mu_static_a2=Brakes.Axle2.DiscAndPad.rMuStatic.Value, brk_mu_kin_a1=Brakes.Axle1.DiscAndPad.rMuKinetic.Value, brk_mu_kin_a2=Brakes.Axle2.DiscAndPad.rMuKinetic.Value, brk_trans_vel_a1=Brakes.Axle1.DiscAndPad.nTransition.Value, brk_trans_vel_a2=Brakes.Axle2.DiscAndPad.nTransition.Value, brk_visc_coef_a1=Brakes.Axle1.DiscAndPad.dViscous.Value, brk_visc_coef_a2=Brakes.Axle2.DiscAndPad.dViscous.Value, brk_max_p_a1=Brakes.Axle1.Caliper.pMax.Value, brk_max_p_a2=Brakes.Axle2.Caliper.pMax.Value, brk_filt_a1=1/Brakes.Axle1.Caliper.fActuatorCutoff.Value, brk_filt_a2=1/Brakes.Axle2.Caliper.fActuatorCutoff.Value}
      mask help: Model braking system with disc brakes for two axles. Takes brake pedal travel as input, actuator dynamics modeled as a transfer function.
      mask TypeOptions brk_pad_rad_a1:
      | Disc
      | Brake
      | L1/r_mean | Disc
      | Brake
      | R1/r_mean
      mask TypeOptions brk_pad_rad_a2:
      | Disc
      | Brake
      | L2/r_mean | Disc
      | Brake
      | R2/r_mean
      mask TypeOptions brk_cyl_bore_a1:
      | Disc
      | Brake
      | L1/bore | Disc
      | Brake
      | R1/bore
      mask TypeOptions brk_cyl_bore_a2:
      | Disc
      | Brake
      | L2/bore | Disc
      | Brake
      | R2/bore
      mask TypeOptions brk_n_pads_a1:
      | Disc
      | Brake
      | L1/n_pads | Disc
      | Brake
      | R1/n_pads
      mask TypeOptions brk_n_pads_a2:
      | Disc
      | Brake
      | L2/n_pads | Disc
      | Brake
      | R2/n_pads
      mask TypeOptions brk_mu_static_a1:
      | Disc
      | Brake
      | L1/mu_static | Disc
      | Brake
      | R1/mu_static
      mask TypeOptions brk_mu_static_a2:
      | Disc
      | Brake
      | L2/mu_static | Disc
      | Brake
      | R2/mu_static
      mask TypeOptions brk_mu_kin_a1:
      | Disc
      | Brake
      | L1/mu_coulomb | Disc
      | Brake
      | R1/mu_coulomb
      mask TypeOptions brk_mu_kin_a2:
      | Disc
      | Brake
      | L2/mu_coulomb | Disc
      | Brake
      | R2/mu_coulomb
      mask TypeOptions brk_trans_vel_a1:
      | Disc
      | Brake
      | L1/brkwy_vel | Disc
      | Brake
      | R1/brkwy_vel
      mask TypeOptions brk_trans_vel_a2:
      | Disc
      | Brake
      | L2/brkwy_vel | Disc
      | Brake
      | R2/brkwy_vel
      mask TypeOptions brk_visc_coef_a1:
      | Disc
      | Brake
      | L1/visc_coef | Disc
      | Brake
      | R1/visc_coef
      mask TypeOptions brk_visc_coef_a2:
      | Disc
      | Brake
      | L2/visc_coef | Disc
      | Brake
      | R2/visc_coef
      mask TypeOptions brk_max_p_a1: Actuator L1/brk_max_p | Actuator R1/brk_max_p
      mask TypeOptions brk_max_p_a2: Actuator L2/brk_max_p | Actuator R2/brk_max_p
      mask TypeOptions brk_filt_a1: Actuator L1/brk_filt | Actuator R1/brk_filt
      mask TypeOptions brk_filt_a2: Actuator L2/brk_filt | Actuator R2/brk_filt
      mask DialogControl cont_brakes Prompt: Brakes
      mask DialogControl cont_brk_geom Prompt: Geometry
      mask DialogControl text_brakes_a1 Prompt: Axle 1
      mask DialogControl text_brakes_a2 Prompt: Axle 2
      mask DialogControl text_brakes_pad_rad Prompt: Mean Pad Radius (m)
      mask DialogControl text_brakes_cyl_bore Prompt: Cylinder Bore (m)
      mask DialogControl text_brakes_n_pads Prompt: Number of pads
      mask DialogControl cont_brk_frict Prompt: Friction
      mask DialogControl text_brakes_mu_static Prompt: Static Coeff. (0-1)
      mask DialogControl text_brakes_mu_kin Prompt: Kinetic Coeff. (0-1)
      mask DialogControl text_brakes_trans_vel Prompt: Trans. Velocity (rad/s)
      mask DialogControl text_brakes_visc_coef Prompt: Viscous (N*m/(rad/s))
      mask DialogControl cont_brk_act Prompt: Actuator
      mask DialogControl text_brakes_maxp Prompt: Max Pad Pressure (Pa)
      mask DialogControl text_brakes_filt Prompt: Time Constant (s)
      mask Display: image('sm_car_vehicle_brakes_pedal_IMAGE.png');
  L1 : PMIOPort  Side=Left
  R1 : PMIOPort  Port=2  Side=Right
  L2 : PMIOPort  Port=3  Side=Left
  R2 : PMIOPort  Port=4  Side=Right
  " OutB" : Outport  VectorParamsAs1DForOutWhenUnconnected=off

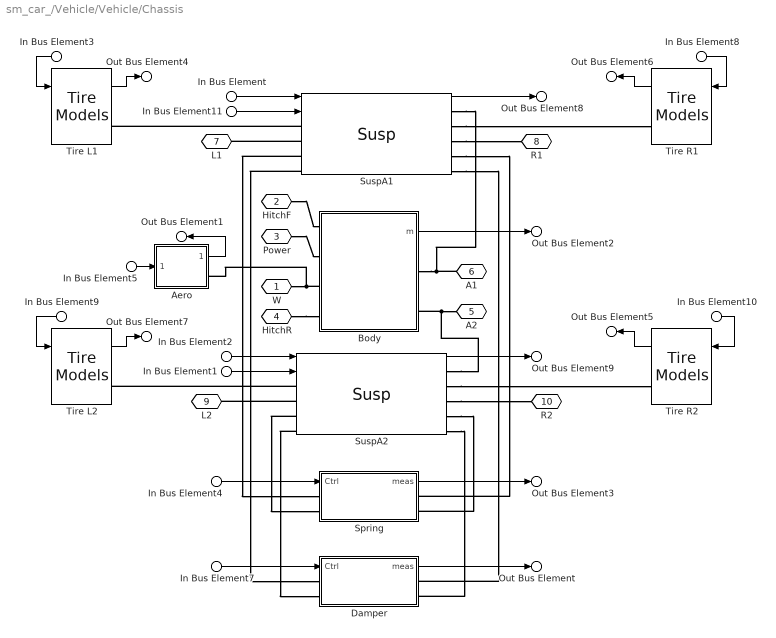
== system sm_car_/Vehicle/Vehicle/Chassis ==
  In Bus Element11 : Inport  PortName=DrvBus
  In Bus Element1 : Inport  PortName=DrvBus
  In Bus Element3 : Inport  Port=2  PortName=RdBus  Element=L1
  In Bus Element8 : Inport  Port=2  PortName=RdBus  Element=R1
  In Bus Element10 : Inport  Port=2  PortName=RdBus  Element=R2
  In Bus Element9 : Inport  Port=2  PortName=RdBus  Element=L2
  In Bus Element5 : Inport  Port=2  PortName=RdBus  Element=fWindCar
  In Bus Element7 : Inport  Port=3  PortName=CtrlBus  Element=Damper
  In Bus Element : Inport  Port=3  PortName=CtrlBus  Element=SuspA1
  In Bus Element4 : Inport  Port=3  PortName=CtrlBus  Element=Spring
  In Bus Element2 : Inport  Port=3  PortName=CtrlBus  Element=SuspA2
  Aero : Subsystem  mask(Aerodynamic Load (Drag, Lift)){CL=Chassis.Aero.CL.Value, CD=Chassis.Aero.CD.Value, rho=Chassis.Aero.rho_air.Value, A=Chassis.Aero.ARef.Value, sCentreOfPressure=Chassis.Aero.sPressureCentre.Value, clr_hp=Visual.hp.clr, opc_hp=Visual.hp.opc, rad_hp=Visual.hp.rad}
      mask prompts: CL "Lift Coeff (-)"; CD "Drag Coeff (-)"; rho "Air Density (kg/m^3)"; A "Reference Area (m^2)"; sCentreOfPressure "Centre of Pressure [xyz] (m)"; clr_hp "Color [RGB]"; opc_hp "Opacity (0-1)"; rad_hp "Radius (m)"
      mask help: Models lift and drag on vehicle.
      mask TypeOptions clr_hp:
      | Vis
      | Center of Pressure/GraphicDiffuseColor
      mask TypeOptions opc_hp:
      | Vis
      | Center of Pressure/GraphicOpacity
      mask TypeOptions rad_hp:
      | Vis
      | Center of Pressure/SphereRadius
      mask DialogControl conv_vis Prompt: Visualization
  Body : Subsystem  mask(Body){hp_mount_a1=Chassis.Body.sAxle1.Value, hp_mount_a2=Chassis.Body.sAxle2.Value, hp_mount_power=Chassis.Body.sPower.Value, hp_chassis_cg=Chassis.Body.sCG.Value, hp_mount_hitchf=Chassis.Body.sHitchF.Value, hp_mount_hitchr=Chassis.Body.sHitchR.Value, chassis_mass=Chassis.Body.m.Value, chassis_inertia=Chassis.Body.J.Value, clr_chassis_hp_cg=Visual.hp.clr, opc_chassis_hp_cg=Visual.hp.opc, size_chassis_hp_cg=Visual.hp.rad, BodyGeometry=Chassis.Body.BodyGeometry, BodyLoad=Chassis.Body.BodyLoad}
      mask prompts: hp_mount_power "HP Power [xyz] (m)"; hp_chassis_cg "Chassis CG [xyz] (m)"; hp_mount_hitchf "Hitch Front [xyz] (m)"; hp_mount_hitchr "Hitch Rear [xyz] (m)"; chassis_mass "Mass (kg)"; chassis_inertia "Inertia [Ixx Iyy Izz]"; BodyGeometry "BodyGeometry (structure)"; BodyLoad "BodyLoad (structure)"
      mask help: Vehicle body mass, inertia, and geometry.
      mask TypeOptions hp_mount_a1:
      | Transform
      | Mount A1/TranslationCartesianOffset
      mask TypeOptions hp_mount_a2:
      | Transform
      | Mount A2/TranslationCartesianOffset
      mask TypeOptions hp_mount_power:
      | Transform
      | Power Mount/TranslationCartesianOffset
      mask TypeOptions hp_chassis_cg:
      | Transform
      | Body CG/TranslationCartesianOffset
      mask TypeOptions hp_mount_hitchf:
      | Transform
      | Front Hitch/TranslationCartesianOffset
      mask TypeOptions hp_mount_hitchr:
      | Transform
      | Rear Hitch/TranslationCartesianOffset
      mask TypeOptions chassis_mass:
      | Body Mass
      | and Inertia/Mass
      mask TypeOptions chassis_inertia:
      | Body Mass
      | and Inertia/MomentsOfInertia
      mask TypeOptions clr_chassis_hp_cg:
      | Body Mass
      | and Inertia/GraphicDiffuseColor | Vis HP Mount A1/GraphicDiffuseColor | Vis HP Hitch/GraphicDiffuseColor
      mask TypeOptions opc_chassis_hp_cg:
      | Body Mass
      | and Inertia/GraphicOpacity | Vis HP Mount A1/GraphicOpacity | Vis HP Hitch/GraphicOpacity
      mask TypeOptions size_chassis_hp_cg:
      | Body Mass
      | and Inertia/SphereRadius | Vis HP Mount A1/SphereRadius | Vis HP Hitch/SphereRadius
      mask DialogControl cont_chassis Prompt: Chassis
      mask DialogControl text_chassis_mount_hp_blank Prompt: [xyz] (m)
      mask DialogControl text_chassis_a1 Prompt: Axle 1
      mask DialogControl text_chassis_a2 Prompt: Axle 2
      mask DialogControl text_chassis_hp_mount Prompt: HP Mount
      mask DialogControl cont_chassis_vis Prompt: Visualization
      mask DialogControl text_chassis_vis_clr Prompt: Color [RGB]
      mask DialogControl text_chassis_vis_opc Prompt: Opacity (0-1)
      mask DialogControl text_chassis_vis_size Prompt: Size [xyz] (m)
      mask DialogControl text_chassis_vis_hp Prompt: Hardpoints
      mask DialogControl cont_body_geometry Prompt: Body
      mask Display:
      | % Get image from BodyGeometry.class
      | % (active choice for Body Geometry subsystem)
      | temp_veh_bg_class = lower(get_param([gcb '/Body Geometry'],'LabelModeActiveChoice'));
      | 
      | imagestr = (['sm_car_body_' temp_veh_bg_class '.png']);
      | if(~exist(imagestr))
      |     imagestr = ['sm_car_body_default.png'];
      | end
      | 
      | image(imagestr);
  Damper : Subsystem  Tag=PublishSubsystem  Variant=on  VariantControlMode=label  VariantControl=Variant1  LabelModeActiveChoice=Independent  mask(Variants for Dampers){Damper=Chassis.Damper, VariantLabel=Chassis.Damper.class.Value}
      mask prompts: Damper "Damper Parameters"; VariantLabel "Variant Label"
      mask help: Select option and provide parameters for left and right dampers on two axles. Option is chosen by string provided in Variant Label. The parameters for the selected option is contained in Dampers data structure.
      mask init:
      | curblk = gcb;
      | 
      | % Set variant for this block 
      | set_param(curblk,'LabelModeActiveChoice',VariantLabel);
      settings: AttributesFormatString=%<ActiveVariant>
      mask Display:
      | if(strcmp(get_param(gcb,'LabelModeActiveChoice'),'None'))
      |     disp(' ');
      | else
      |     image('sm_car_vehicle_chassis_damper_IMAGE.png');
      | end
  Spring : Subsystem  Tag=PublishSubsystem  Variant=on  VariantControlMode=label  VariantControl=Variant1  LabelModeActiveChoice=Independent  mask(Variants for Springs){Spring=Chassis.Spring, VariantLabel=Chassis.Spring.class.Value}
      mask prompts: Spring "Spring Parameters"; VariantLabel "Variant Label"
      mask help: Select option and provide parameters for left and right springs on two axles. Option is chosen by string provided in Variant Label. The parameters for the selected option is contained in Springs data structure.
      mask init:
      | curblk = gcb;
      | 
      | % Set variant for this block 
      | set_param(curblk,'LabelModeActiveChoice',VariantLabel);
      settings: AttributesFormatString=%<ActiveVariant>
      mask Display:
      | if(strcmp(get_param(gcb,'LabelModeActiveChoice'),'None'))
      |     disp(' ');
      | else
      |     image('sm_car_vehicle_chassis_spring_IMAGE.png');
      | end
  SuspA1 : Linkage/Susp  VariantControl=Variant1  LabelModeActiveChoice=Linkage  Susp=Chassis.SuspA1  Init=Init.Axle1  VariantLabel=Chassis.SuspA1.class.Value
      link override Linkage/Steer/Wheel Driven Rack 1UJoint: len_sha_u=Steer.Shaft_Upper.xLength.Value
      settings: AttributesFormatString=%<LabelModeActiveChoice>
  SuspA2 : Linkage/Susp  VariantControl=Variant1  LabelModeActiveChoice=Linkage  Susp=Chassis.SuspA2  Init=Init.Axle2  VariantLabel=Chassis.SuspA2.class.Value
      settings: AttributesFormatString=%<LabelModeActiveChoice>
  Tire L1 : Tire_1x2x/Tire Models  Tag=PublishSubsystem  VariantControl=Variant1  LabelModeActiveChoice=MFEval  popup_leftRight=Left  tir_index=veh_index  Tire=Chassis.Tire  VariantLabel=Chassis.Tire.class.Value
      settings: AttributesFormatString=%<ActiveVariant>
  Tire L2 : Tire_1x2x/Tire Models  Tag=PublishSubsystem  VariantControl=Variant1  LabelModeActiveChoice=MFEval  popup_leftRight=Left  tir_index=veh_index+10  Tire=Chassis.Tire  VariantLabel=Chassis.Tire.class.Value
      settings: AttributesFormatString=%<ActiveVariant>
  Tire R1 : Tire_1x2x/Tire Models  Tag=PublishSubsystem  VariantControl=Variant1  LabelModeActiveChoice=MFEval  popup_leftRight=Right  tir_index=veh_index+4  Tire=Chassis.Tire  VariantLabel=Chassis.Tire.class.Value
      settings: AttributesFormatString=%<ActiveVariant>
  Tire R2 : Tire_1x2x/Tire Models  Tag=PublishSubsystem  VariantControl=Variant1  LabelModeActiveChoice=MFEval  popup_leftRight=Right  tir_index=veh_index+14  Tire=Chassis.Tire  VariantLabel=Chassis.Tire.class.Value
      settings: AttributesFormatString=%<ActiveVariant>
  W : PMIOPort  Side=Right
  HitchF : PMIOPort  Port=2  Side=Right
  Power : PMIOPort  Port=3  Side=Right
  HitchR : PMIOPort  Port=4  Side=Left
  A2 : PMIOPort  Port=5  Side=Right
  A1 : PMIOPort  Port=6  Side=Left
  L1 : PMIOPort  Port=7  Side=Left
  R1 : PMIOPort  Port=8  Side=Right
  L2 : PMIOPort  Port=9  Side=Left
  R2 : PMIOPort  Port=10  Side=Right
  Out Bus Element4 : Outport  VectorParamsAs1DForOutWhenUnconnected=off  PortName=VehBus  Element=WhlL1
  Out Bus Element6 : Outport  VectorParamsAs1DForOutWhenUnconnected=off  PortName=VehBus  Element=WhlR1
  Out Bus Element5 : Outport  VectorParamsAs1DForOutWhenUnconnected=off  PortName=VehBus  Element=WhlR2
  Out Bus Element7 : Outport  VectorParamsAs1DForOutWhenUnconnected=off  PortName=VehBus  Element=WhlL2
  Out Bus Element1 : Outport  VectorParamsAs1DForOutWhenUnconnected=off  PortName=VehBus  Element=Aero
  Out Bus Element : Outport  VectorParamsAs1DForOutWhenUnconnected=off  PortName=VehBus  Element=Damper
  Out Bus Element3 : Outport  VectorParamsAs1DForOutWhenUnconnected=off  PortName=VehBus  Element=Spring
  Out Bus Element8 : Outport  VectorParamsAs1DForOutWhenUnconnected=off  PortName=VehBus  Element=SuspA1
  Out Bus Element9 : Outport  VectorParamsAs1DForOutWhenUnconnected=off  PortName=VehBus  Element=SuspA2
  Out Bus Element2 : Outport  VectorParamsAs1DForOutWhenUnconnected=off  PortName=VehBus  Element=Body
  wires:
  Body/1(m) -> Out Bus Element2/1
  In Bus Element5/1 -> Aero/1(fWind)
  Aero/1(meas) -> Out Bus Element1/1
  In Bus Element4/1 -> Spring/1("Ctrl ")
  In Bus Element7/1 -> Damper/1("Ctrl ")
  In Bus Element2/1 -> SuspA2/1
  SuspA2/1 -> Out Bus Element9/1
  In Bus Element1/1 -> SuspA2/2
  In Bus Element/1 -> SuspA1/1
  SuspA1/1 -> Out Bus Element8/1
  In Bus Element11/1 -> SuspA1/2
  Tire R2/1 -> Out Bus Element5/1
  In Bus Element9/1 -> Tire L2/1
  Tire L1/1 -> Out Bus Element4/1
  In Bus Element8/1 -> Tire R1/1
  Tire L2/1 -> Out Bus Element7/1
  In Bus Element10/1 -> Tire R2/1
  Tire R1/1 -> Out Bus Element6/1
  In Bus Element3/1 -> Tire L1/1
  Damper/1(" meas") -> Out Bus Element/1
  Spring/1(" meas") -> Out Bus Element3/1
  connections:
  HitchR/RConn1 -- Body/LConn4
  Power/RConn1 -- Body/LConn2
  SuspA2/RConn5 -- Damper/RConn2
  SuspA2/LConn4 -- Damper/LConn2
  SuspA2/RConn4 -- Spring/RConn2
  SuspA2/LConn3 -- Spring/LConn2
  SuspA2/RConn3 -- R2/RConn1
  SuspA2/LConn2 -- L2/RConn1
  SuspA2/RConn2 -- Tire R2/RConn1
  SuspA2/LConn1 -- Tire L2/RConn1
  SuspA1/RConn5 -- Damper/RConn1
  SuspA1/LConn4 -- Damper/LConn1
  SuspA1/RConn4 -- Spring/RConn1
  SuspA1/LConn3 -- Spring/LConn1
  Body/RConn1 -- SuspA1/RConn1 -- A1/RConn1
  SuspA1/LConn1 -- Tire L1/RConn1
  SuspA1/RConn2 -- Tire R1/RConn1
  SuspA1/RConn3 -- R1/RConn1
  SuspA1/LConn2 -- L1/RConn1
  SuspA2/RConn1 -- A2/RConn1 -- Body/RConn2
  W/RConn1 -- Body/LConn3 -- Aero/RConn1
  HitchF/RConn1 -- Body/LConn1
